simulink library "lib_imuCal"  (Simulink 9.0)
settings: Solver=VariableStepAuto  StartTime=0.0  StopTime=10.0  RelTol=1e-3
undefined symbols (not defined in the file): g, toa_imuBasicOrient
libraries: lib_CATutils_Utilities_ApplyName_v2 x14, lib_imuCal x2, simulink_extras x2, lib_CATutils_Override x2
(part 1 of 2)
settings Model: Creator=currisd  LastModifiedBy=CurriSD

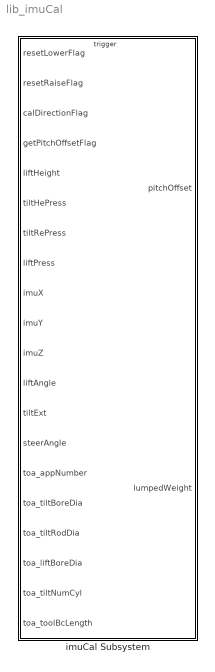
== system lib_imuCal ==
  imuCal Subsystem : Subsystem

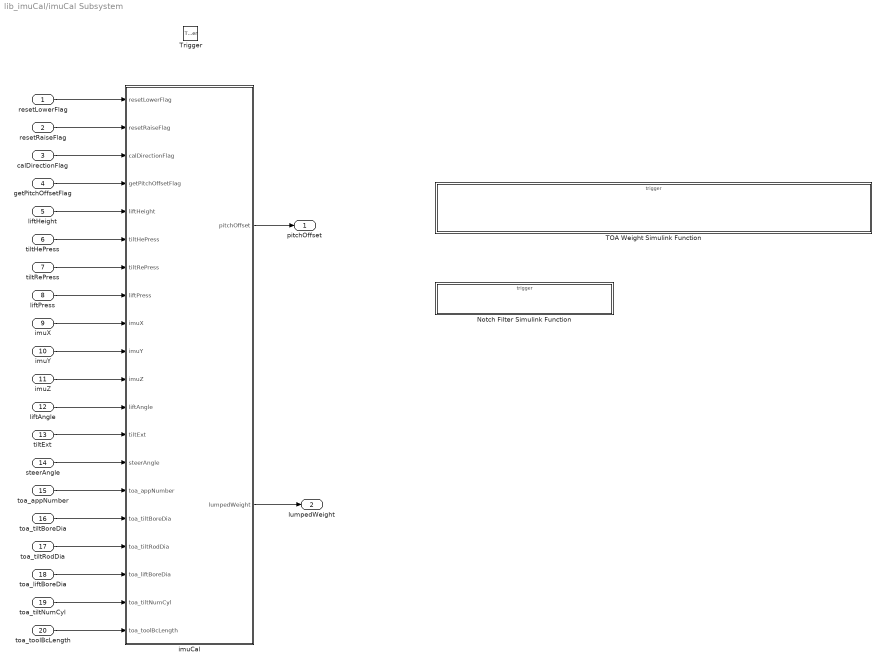
== system lib_imuCal/imuCal Subsystem ==
  resetLowerFlag : Inport
  resetRaiseFlag : Inport  Port=2
  calDirectionFlag : Inport  Port=3
  getPitchOffsetFlag : Inport  Port=4
  liftHeight : Inport  Port=5
  tiltHePress : Inport  Port=6
  tiltRePress : Inport  Port=7
  liftPress : Inport  Port=8
  imuX : Inport  Port=9
  imuY : Inport  Port=10
  imuZ : Inport  Port=11
  liftAngle : Inport  Port=12
  tiltExt : Inport  Port=13
  steerAngle : Inport  Port=14
  toa_appNumber : Inport  Port=15
  toa_tiltBoreDia : Inport  Port=16
  toa_tiltRodDia : Inport  Port=17
  toa_liftBoreDia : Inport  Port=18
  toa_tiltNumCyl : Inport  Port=19
  toa_toolBcLength : Inport  Port=20
  Trigger : TriggerPort  TriggerType=function-call  FunctionName=imuCalWrapper  FunctionVisibility=scoped  VariantControl=Variant  PortDimensions=1
  Notch Filter Simulink Function : Subsystem
  TOA Weight Simulink Function : Subsystem  TreatAsAtomicUnit=on
      settings: PropExecContextOutsideSubsystem=on
  imuCal : MATLAB Function  TreatAsAtomicUnit=on
  pitchOffset : Outport
  lumpedWeight : Outport  Port=2
  wires:
  tiltHePress/1 -> imuCal/6(tiltHePress)
  steerAngle/1 -> imuCal/14(steerAngle)
  liftHeight/1 -> imuCal/5(liftHeight)
  tiltRePress/1 -> imuCal/7(tiltRePress)
  liftPress/1 -> imuCal/8(liftPress)
  tiltExt/1 -> imuCal/13(tiltExt)
  imuZ/1 -> imuCal/11(imuZ)
  liftAngle/1 -> imuCal/12(liftAngle)
  imuX/1 -> imuCal/9(imuX)
  imuY/1 -> imuCal/10(imuY)
  resetLowerFlag/1 -> imuCal/1(resetLowerFlag)
  calDirectionFlag/1 -> imuCal/3(calDirectionFlag)
  resetRaiseFlag/1 -> imuCal/2(resetRaiseFlag)
  getPitchOffsetFlag/1 -> imuCal/4(getPitchOffsetFlag)
  imuCal/1(pitchOffset) -> pitchOffset/1
  toa_appNumber/1 -> imuCal/15(toa_appNumber)
  toa_tiltBoreDia/1 -> imuCal/16(toa_tiltBoreDia)
  toa_tiltRodDia/1 -> imuCal/17(toa_tiltRodDia)
  toa_liftBoreDia/1 -> imuCal/18(toa_liftBoreDia)
  toa_tiltNumCyl/1 -> imuCal/19(toa_tiltNumCyl)
  toa_toolBcLength/1 -> imuCal/20(toa_toolBcLength)
  imuCal/2(lumpedWeight) -> lumpedWeight/1

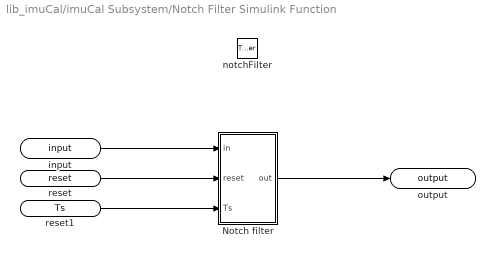
== system lib_imuCal/imuCal Subsystem/Notch Filter Simulink Function ==
  notchFilter : TriggerPort  TriggerType=function-call  IsSimulinkFunction=on  FunctionName=notchFilter  FunctionVisibility=scoped  VariantControl=Variant  PortDimensions=1
  Notch filter : Subsystem
  input : ArgIn  OutDataTypeStr=single  ArgumentName=input
  reset : ArgIn  Port=2  OutDataTypeStr=boolean  ArgumentName=reset
  reset1 : ArgIn  Port=3  OutDataTypeStr=single  ArgumentName=Ts
  output : ArgOut  OutDataTypeStr=single  ArgumentName=output
  wires:
  input/1 -> Notch filter/1(in)
  reset/1 -> Notch filter/2(reset)
  Notch filter/1(out) -> output/1
  reset1/1 -> Notch filter/3(Ts)

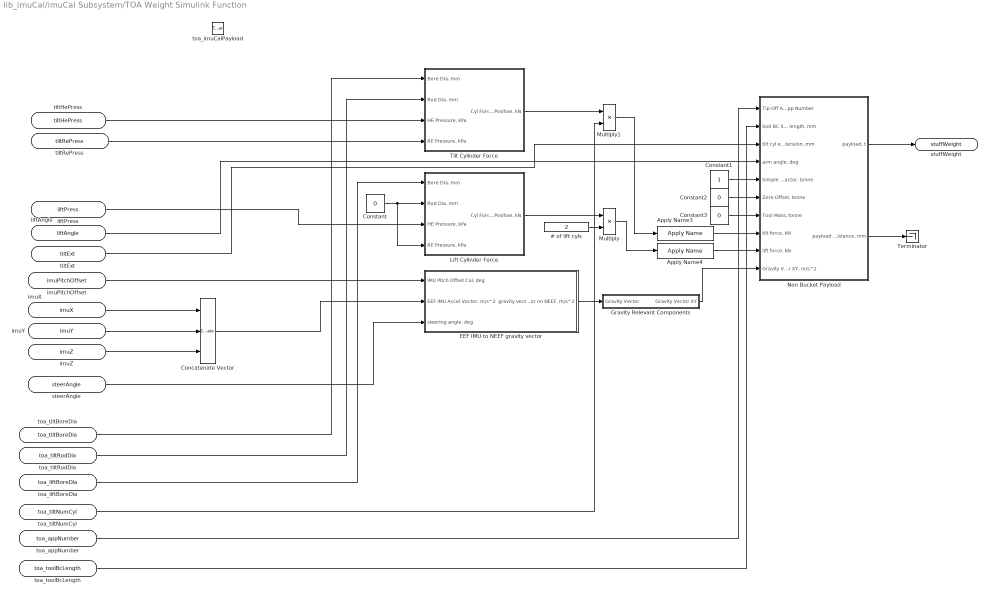
== system lib_imuCal/imuCal Subsystem/TOA Weight Simulink Function ==
  toa_imuCalPayload : TriggerPort  TriggerType=function-call  IsSimulinkFunction=on  FunctionName=toa_imuCalPayload  FunctionVisibility=scoped  VariantControl=(inherit)
  # of lift cyls : Constant  Value=2  OutDataTypeStr=single
  Apply Name3 : lib_CATutils_Utilities_ApplyName_v2/Apply Name  sigLabel='toa_tiltForce'  enTst=true
  Apply Name4 : lib_CATutils_Utilities_ApplyName_v2/Apply Name  sigLabel='toa_liftForce'  enTst=true
  Concatenate Vector : Concatenate  NumInputs=3  Mode=Multidimensional array
  Constant : Constant  Value=0  OutDataTypeStr=Inherit: Inherit via back propagation
  Constant1 : Constant  OutDataTypeStr=single
  Constant2 : Constant  Value=0  OutDataTypeStr=Inherit: Inherit via back propagation
  Constant3 : Constant  Value=0  OutDataTypeStr=Inherit: Inherit via back propagation
  EEF IMU to NEEF gravity vector : Subsystem
  Gravity Relevant Components : Subsystem
  Lift Cylinder Force : Subsystem
  Multiply : Product  SaturateOnIntegerOverflow=on  RndMeth=Zero  InputSameDT=on  OutDataTypeStr=Inherit: Same as first input
  Multiply1 : Product  OutDataTypeStr=single  SaturateOnIntegerOverflow=on  RndMeth=Zero
  Non Bucket Payload : Subsystem
  Terminator : Terminator
  Tilt Cylinder Force : Subsystem
  liftAngle : ArgIn  DisableCoverage=on  OutDataTypeStr=single  ArgumentName=liftAngle
  tiltExt : ArgIn  DisableCoverage=on  Port=2  OutDataTypeStr=single  ArgumentName=tiltExt
  tiltHePress : ArgIn  DisableCoverage=on  Port=3  OutDataTypeStr=single  ArgumentName=tiltHePress
  tiltRePress : ArgIn  DisableCoverage=on  Port=4  OutDataTypeStr=single  ArgumentName=tiltRePress
  liftPress : ArgIn  DisableCoverage=on  Port=5  OutDataTypeStr=single  ArgumentName=liftPress
  imuX : ArgIn  DisableCoverage=on  Port=6  OutDataTypeStr=single  ArgumentName=imuX
  imuY : ArgIn  DisableCoverage=on  Port=7  OutDataTypeStr=single  ArgumentName=imuY
  imuZ : ArgIn  DisableCoverage=on  Port=8  OutDataTypeStr=single  ArgumentName=imuZ
  steerAngle : ArgIn  DisableCoverage=on  Port=9  OutDataTypeStr=single  ArgumentName=steerAngle
  imuPitchOffset : ArgIn  Port=10  OutDataTypeStr=single  ArgumentName=imuPitchOffset
  toa_appNumber : ArgIn  Port=11  OutDataTypeStr=uint32  ArgumentName=toa_appNumber
  toa_tiltBoreDia : ArgIn  Port=12  OutDataTypeStr=single  ArgumentName=toa_tiltBoreDia
  toa_tiltRodDia : ArgIn  Port=13  OutDataTypeStr=single  ArgumentName=toa_tiltRodDia
  toa_liftBoreDia : ArgIn  Port=14  OutDataTypeStr=single  ArgumentName=toa_liftBoreDia
  toa_tiltNumCyl : ArgIn  Port=15  OutDataTypeStr=uint8  ArgumentName=toa_tiltNumCyl
  toa_toolBcLength : ArgIn  Port=16  OutDataTypeStr=single  ArgumentName=toa_toolBcLength
  stuffWeight : ArgOut  DisableCoverage=on  OutDataTypeStr=single  ArgumentName=stuffWeight
  wires:
  Constant2/1 -> Non Bucket Payload/6("Zero Offset, tonne")
  toa_appNumber/1 -> Non Bucket Payload/1(Tip-Off Assist App Number)
  Multiply/1 -> Apply Name4/1
  Multiply1/1 -> Apply Name3/1
  liftAngle/1 -> Non Bucket Payload/4("arm angle, deg")
  # of lift cyls/1 -> Multiply/2
  Constant/1 -> Lift Cylinder Force/4("RE Pressure, kPa"), Lift Cylinder Force/2("Rod Dia, mm")
  Constant1/1 -> Non Bucket Payload/5("Simple Cal Factor, tonne")
  Tilt Cylinder Force/1("Cyl Force, Compression Positive, kN") -> Multiply1/1
  Lift Cylinder Force/1("Cyl Force, Compression Positive, kN") -> Multiply/1
  Apply Name3/1 -> Non Bucket Payload/8("tilt force, kN")
  Apply Name4/1 -> Non Bucket Payload/9("lift force, kN")
  Constant3/1 -> Non Bucket Payload/7("Tool Mass, tonne")
  toa_tiltNumCyl/1 -> Multiply1/2
  Gravity Relevant Components/1(Gravity Vector XY) -> Non Bucket Payload/10("Gravity Vector XY, m/s^2")
  EEF IMU to NEEF gravity vector/1("gravity vector on NEEF, m/s^2") -> Gravity Relevant Components/1(Gravity Vector)
  tiltExt/1 -> Non Bucket Payload/3("tilt cyl extension, mm")
  toa_toolBcLength/1 -> Non Bucket Payload/2("tool BC link length, mm")
  Non Bucket Payload/1("payload, t") -> stuffWeight/1
  Non Bucket Payload/2("payload distance, mm") -> Terminator/1
  toa_tiltBoreDia/1 -> Tilt Cylinder Force/1("Bore Dia, mm")
  toa_tiltRodDia/1 -> Tilt Cylinder Force/2("Rod Dia, mm")
  toa_liftBoreDia/1 -> Lift Cylinder Force/1("Bore Dia, mm")
  tiltHePress/1 -> Tilt Cylinder Force/3("HE Pressure, kPa")
  tiltRePress/1 -> Tilt Cylinder Force/4("RE Pressure, kPa")
  liftPress/1 -> Lift Cylinder Force/3("HE Pressure, kPa")
  imuPitchOffset/1 -> EEF IMU to NEEF gravity vector/1("IMU Pitch Offset Cal, deg")
  Concatenate Vector/1 -> EEF IMU to NEEF gravity vector/2("EEF IMU Accel Vector, m/s^2")
  imuX/1 -> Concatenate Vector/1
  imuY/1 -> Concatenate Vector/2
  imuZ/1 -> Concatenate Vector/3
  steerAngle/1 -> EEF IMU to NEEF gravity vector/3("steering angle, deg")

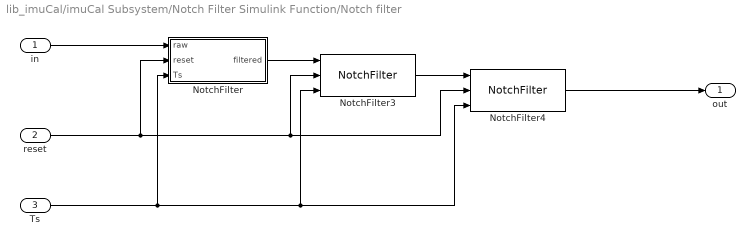
== system lib_imuCal/imuCal Subsystem/Notch Filter Simulink Function/Notch filter ==
  in : Inport
  reset : Inport  Port=2
  Ts : Inport  Port=3
  NotchFilter : Subsystem  mask{mskCutoffFreqRadPerSec=5.0}
      mask prompts: mskCutoffFreqRadPerSec "Cutoff Frequency (rad/s)"
      settings: AttributesFormatString=cf: %<mskCutoffFreqRadPerSec>
  NotchFilter3 : lib_imuCal/imuCal Subsystem/Notch Filter Simulink Function/Notch filter/NotchFilter  mskCutoffFreqRadPerSec=7.5
      settings: AttributesFormatString=cf: %<mskCutoffFreqRadPerSec>
  NotchFilter4 : lib_imuCal/imuCal Subsystem/Notch Filter Simulink Function/Notch filter/NotchFilter  mskCutoffFreqRadPerSec=12
      settings: AttributesFormatString=cf: %<mskCutoffFreqRadPerSec>
  out : Outport
  wires:
  NotchFilter/1(filtered) -> NotchFilter3/1
  NotchFilter3/1 -> NotchFilter4/1
  reset/1 -> NotchFilter3/2, NotchFilter4/2, NotchFilter/2(reset)
  in/1 -> NotchFilter/1(raw)
  NotchFilter4/1 -> out/1
  Ts/1 -> NotchFilter/3(Ts), NotchFilter4/3, NotchFilter3/3

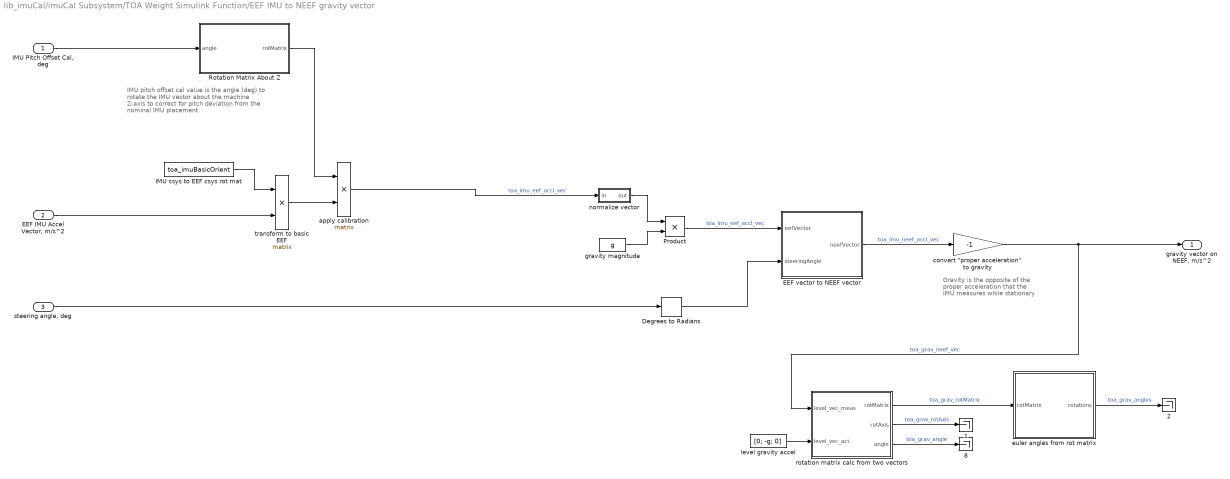
== system lib_imuCal/imuCal Subsystem/TOA Weight Simulink Function/EEF IMU to NEEF gravity vector ==
  note: Gravity is the opposite of the proper acceleration that the IMU measures while stationary
  note: IMU pitch offset cal value is the angle (deg) to rotate the IMU vector about the machine Z-axis to correct for pitch deviation from the nominal IMU placement.
  "IMU Pitch Offset Cal, deg" : Inport
  "EEF IMU Accel Vector, m/s^2" : Inport  Port=2
  "steering angle, deg" : Inport  Port=3
  " 1" : Terminator
  " 2" : Terminator
  " 8" : Terminator
  Degrees to Radians : simulink_extras/Transformations/Degrees to Radians
  EEF vector to NEEF vector : MATLAB Function  TreatAsAtomicUnit=on
  IMU csys to EEF csys rot mat : Constant  Value=toa_imuBasicOrient  VectorParams1D=off  OutDataTypeStr=single  SampleTime=-1
  Product : Product  Inputs=**  OutDataTypeStr=Inherit: Same as first input
  Rotation Matrix About Z : MATLAB Function  TreatAsAtomicUnit=on
  apply calibration : Product  Multiplication=Matrix(*)  SaturateOnIntegerOverflow=on  RndMeth=Zero  OutDataTypeStr=Inherit: Same as first input
  "convert \"proper acceleration\" to gravity" : Gain  Gain=-1  SaturateOnIntegerOverflow=on  OutDataTypeStr=Inherit: Same as input  ParamDataTypeStr=Inherit: Same as input
  euler angles from rot matrix : MATLAB Function  TreatAsAtomicUnit=on
  gravity magnitude : Constant  Value=g  OutDataTypeStr=single  SampleTime=-1
  level gravity accel : Constant  Value=[0; -g; 0]  OutDataTypeStr=single  SampleTime=-1
  normalize vector : Subsystem
  rotation matrix calc from two vectors : MATLAB Function  TreatAsAtomicUnit=on
  transform to basic EEF : Product  Multiplication=Matrix(*)  SaturateOnIntegerOverflow=on  RndMeth=Zero  OutDataTypeStr=Inherit: Same as first input
  "gravity vector on NEEF, m/s^2" : Outport
  wires:
  euler angles from rot matrix/1(rotations) -> " 2"/1  "toa_grav_angles"
  Degrees to Radians/1 -> EEF vector to NEEF vector/2(steeringAngle)
  Product/1 -> EEF vector to NEEF vector/1(eefVector)  "toa_imu_eef_accl_vec"
  "steering angle, deg"/1 -> Degrees to Radians/1
  EEF vector to NEEF vector/1(neefVector) -> "convert \"proper acceleration\" to gravity"/1  "toa_imu_neef_accl_vec"
  normalize vector/1(out) -> Product/1
  gravity magnitude/1 -> Product/2
  "IMU Pitch Offset Cal, deg"/1 -> Rotation Matrix About Z/1(angle)
  Rotation Matrix About Z/1(rotMatrix) -> apply calibration/1
  apply calibration/1 -> normalize vector/1(in)  "toa_imu_eef_accl_vec"
  transform to basic EEF/1 -> apply calibration/2
  IMU csys to EEF csys rot mat/1 -> transform to basic EEF/1
  "convert \"proper acceleration\" to gravity"/1 -> rotation matrix calc from two vectors/1(level_vec_meas), "gravity vector on NEEF, m/s^2"/1  "toa_grav_neef_vec"
  "EEF IMU Accel Vector, m/s^2"/1 -> transform to basic EEF/2
  rotation matrix calc from two vectors/1(rotMatrix) -> euler angles from rot matrix/1(rotMatrix)  "toa_grav_rotMatrix"
  rotation matrix calc from two vectors/2(rotAxis) -> " 1"/1  "toa_grav_rotAxis"
  rotation matrix calc from two vectors/3(angle) -> " 8"/1  "toa_grav_angle"
  level gravity accel/1 -> rotation matrix calc from two vectors/2(level_vec_act)

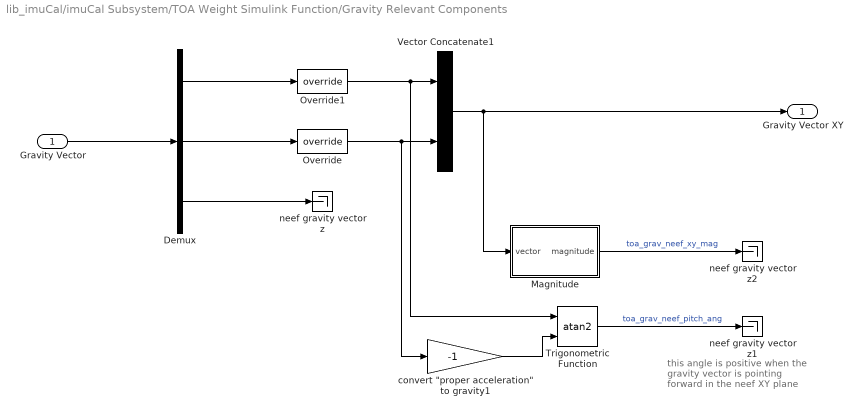
== system lib_imuCal/imuCal Subsystem/TOA Weight Simulink Function/Gravity Relevant Components ==
  note: this angle is positive when the gravity vector is pointing forward in the neef XY plane
  Gravity Vector : Inport
  " neef gravity vector z" : Terminator
  " neef gravity vector z1" : Terminator
  " neef gravity vector z2" : Terminator
  Demux : Demux  Outputs=3
  Magnitude : Subsystem
  Override : lib_CATutils_Override/override  ovType=OV if OV ~= Pass  extOV=off  ov_value=toa_grav_y_ov_val  extPass=off  pass_value=0  extRange=off  ov_max=100  ov_min=1  extCond=off  ov_cond=0  extTF=off  ov_TrueComp=1  ov_FalseComp=2
  Override1 : lib_CATutils_Override/override  ovType=OV if OV ~= Pass  extOV=off  ov_value=toa_grav_x_ov_val  extPass=off  pass_value=0  extRange=off  ov_max=100  ov_min=1  extCond=off  ov_cond=0  extTF=off  ov_TrueComp=1  ov_FalseComp=2
  Trigonometric Function : Trigonometry  Operator=atan2  OutputSignalType=real
  Vector Concatenate1 : Concatenate  Mode=Multidimensional array
  "convert \"proper acceleration\" to gravity1" : Gain  Gain=-1  SaturateOnIntegerOverflow=on  OutDataTypeStr=Inherit: Same as input  ParamDataTypeStr=Inherit: Same as input
  Gravity Vector XY : Outport
  wires:
  Gravity Vector/1 -> Demux/1
  Override/1 -> "convert \"proper acceleration\" to gravity1"/1, Vector Concatenate1/2
  Override1/1 -> Trigonometric Function/1, Vector Concatenate1/1
  Magnitude/1(magnitude) -> " neef gravity vector z2"/1  "toa_grav_neef_xy_mag"
  Trigonometric Function/1 -> " neef gravity vector z1"/1  "toa_grav_neef_pitch_ang"
  "convert \"proper acceleration\" to gravity1"/1 -> Trigonometric Function/2
  Demux/3 -> " neef gravity vector z"/1
  Demux/2 -> Override/1
  Demux/1 -> Override1/1
  Vector Concatenate1/1 -> Magnitude/1(vector), Gravity Vector XY/1

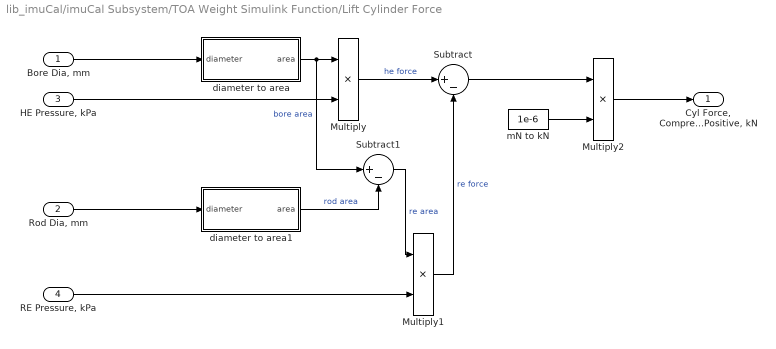
== system lib_imuCal/imuCal Subsystem/TOA Weight Simulink Function/Lift Cylinder Force ==
  "Bore Dia, mm" : Inport
  "Rod Dia, mm" : Inport  Port=2
  "HE Pressure, kPa" : Inport  Port=3
  "RE Pressure, kPa" : Inport  Port=4
  Multiply : Product  SaturateOnIntegerOverflow=on  RndMeth=Zero  InputSameDT=on  OutDataTypeStr=Inherit: Same as first input
  Multiply1 : Product  SaturateOnIntegerOverflow=on  RndMeth=Zero  InputSameDT=on  OutDataTypeStr=Inherit: Same as first input
  Multiply2 : Product  SaturateOnIntegerOverflow=on  RndMeth=Zero  InputSameDT=on  OutDataTypeStr=Inherit: Same as first input
  Subtract : Sum  Inputs=|+-  SaturateOnIntegerOverflow=on  InputSameDT=on  OutDataTypeStr=Inherit: Same as first input
  Subtract1 : Sum  Inputs=|+-  SaturateOnIntegerOverflow=on  InputSameDT=on  OutDataTypeStr=Inherit: Same as first input
  diameter to area : Subsystem
  diameter to area1 : Subsystem
  mN to kN : Constant  Value=1e-6  OutDataTypeStr=single
  "Cyl Force, Compression Positive, kN" : Outport
  wires:
  "HE Pressure, kPa"/1 -> Multiply/2
  Subtract/1 -> Multiply2/1
  "Bore Dia, mm"/1 -> diameter to area/1(diameter)
  Multiply1/1 -> Subtract/2  "re force"
  Multiply/1 -> Subtract/1  "he force"
  diameter to area/1(area) -> Subtract1/1, Multiply/1  "bore area"
  diameter to area1/1(area) -> Subtract1/2  "rod area"
  "RE Pressure, kPa"/1 -> Multiply1/2
  "Rod Dia, mm"/1 -> diameter to area1/1(diameter)
  Subtract1/1 -> Multiply1/1  "re area"
  mN to kN/1 -> Multiply2/2
  Multiply2/1 -> "Cyl Force, Compression Positive, kN"/1

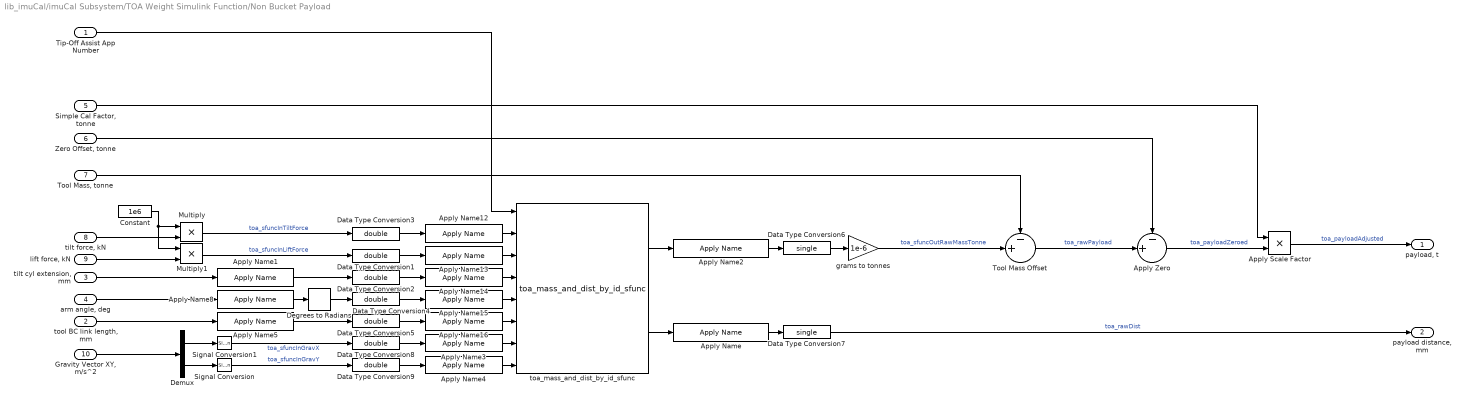
== system lib_imuCal/imuCal Subsystem/TOA Weight Simulink Function/Non Bucket Payload ==
  Tip-Off Assist App Number : Inport
  "tool BC link length, mm" : Inport  Port=2
  "tilt cyl extension, mm" : Inport  Port=3
  "arm angle, deg" : Inport  Port=4
  "Simple Cal Factor, tonne" : Inport  Port=5
  "Zero Offset, tonne" : Inport  Port=6
  "Tool Mass, tonne" : Inport  Port=7
  "tilt force, kN" : Inport  Port=8
  "lift force, kN" : Inport  Port=9
  "Gravity Vector XY, m/s^2" : Inport  Port=10
  Apply Name : lib_CATutils_Utilities_ApplyName_v2/Apply Name  sigLabel='toa_sfuncOutRawDist'  enTst=true
  Apply Name1 : lib_CATutils_Utilities_ApplyName_v2/Apply Name  sigLabel='toa_sfuncInTiltExt'  enTst=true
  Apply Name12 : lib_CATutils_Utilities_ApplyName_v2/Apply Name  sigLabel='toa_sfuncInRawTiltForce'  enTst=true
  Apply Name13 : lib_CATutils_Utilities_ApplyName_v2/Apply Name  sigLabel='toa_sfuncInRawLiftForce'  enTst=true
  Apply Name14 : lib_CATutils_Utilities_ApplyName_v2/Apply Name  sigLabel='toa_sfuncInRawTiltExt'  enTst=true
  Apply Name15 : lib_CATutils_Utilities_ApplyName_v2/Apply Name  sigLabel='toa_sfuncInRawLiftAng'  enTst=true
  Apply Name16 : lib_CATutils_Utilities_ApplyName_v2/Apply Name  sigLabel='toa_sfuncInRawBcLength'  enTst=true
  Apply Name2 : lib_CATutils_Utilities_ApplyName_v2/Apply Name  sigLabel='toa_sfuncOutRawMass'  enTst=true
  Apply Name3 : lib_CATutils_Utilities_ApplyName_v2/Apply Name  sigLabel='toa_sfuncInRawGravX'  enTst=true
  Apply Name4 : lib_CATutils_Utilities_ApplyName_v2/Apply Name  sigLabel='toa_sfuncInRawGravY'  enTst=true
  Apply Name5 : lib_CATutils_Utilities_ApplyName_v2/Apply Name  sigLabel='toa_sfuncInBcLength'  enTst=true
  Apply Name8 : lib_CATutils_Utilities_ApplyName_v2/Apply Name  sigLabel='toa_sfuncInLiftAng'  enTst=true
  Apply Scale Factor : Product
  Apply Zero : Sum  Inputs=-+|  SaturateOnIntegerOverflow=on  InputSameDT=on  OutDataTypeStr=Inherit: Same as first input
  Constant : Constant  Value=1e6  OutDataTypeStr=single
  Data Type Conversion{1..5,8..9} (7 alike) : DataTypeConversion  OutDataTypeStr=double  SaturateOnIntegerOverflow=on  RndMeth=Zero
      settings: AttributesFormatString=Output Data Type: %<OutDataTypeStr>\n
  Data Type Conversion6 : DataTypeConversion  OutDataTypeStr=single  SaturateOnIntegerOverflow=on  RndMeth=Zero
      settings: AttributesFormatString=Output Data Type: %<OutDataTypeStr>\n
  Data Type Conversion7 : DataTypeConversion  OutDataTypeStr=single  SaturateOnIntegerOverflow=on  RndMeth=Zero
      settings: AttributesFormatString=Output Data Type: %<OutDataTypeStr>\n
  Degrees to Radians : simulink_extras/Transformations/Degrees to Radians
  Demux : Demux  Outputs=2
  Multiply : Product  SaturateOnIntegerOverflow=on  RndMeth=Zero  InputSameDT=on  OutDataTypeStr=Inherit: Same as first input
  Multiply1 : Product  SaturateOnIntegerOverflow=on  RndMeth=Zero  InputSameDT=on  OutDataTypeStr=Inherit: Same as first input
  Signal Conversion : SignalConversion  OverrideOpt=on
  Signal Conversion1 : SignalConversion  OverrideOpt=on
  Tool Mass Offset : Sum  Inputs=-+|  SaturateOnIntegerOverflow=on  InputSameDT=on  OutDataTypeStr=Inherit: Same as first input
  grams to tonnes : Gain  Gain=1e-6  SaturateOnIntegerOverflow=on  OutDataTypeStr=Inherit: Same as input  ParamDataTypeStr=Inherit: Same as input
  toa_mass_and_dist_by_id_sfunc : S-Function  FunctionName=toa_mass_and_dist_by_id_sfunc  SFunctionDeploymentMode=off  EnableBusSupport=off  mask(Legacy Function){SFunctionSpec=void toa_mass_and_dist_by_id(uint32 u1, double u2, double u3, double u4, double u5, double u6, double u7, double u8, double y1[1], double y2[1]), ShowSpec=off}
      mask prompts: ShowSpec "Display function specification"
      mask help:
      | This block allows you to call the legacy functions specified by the following Legacy Code Tool definition:
      | def.SFunctionName = 'toa_mass_and_dist_by_id_sfunc';
      | def.OutputFcnSpec = 'void toa_mass_and_dist_by_id(uint32 u1, double u2, double u3, double u4, double u5, double u6, double u7, double u8, double y1[1], double y2[1])';
      | def.HeaderFiles = {'tipoff_assist.h'};
      | def.SourceFiles = {'tipoff_assist.c'};
      | def.IncPaths = {'./c_src'};
      mask Help: <p>This block was generated automatically by the Legacy Code Tool. For detailed help on this tool, call<a href="matlab:legacy_code('help')"> legacy_code('help')</a>.</p>
      mask Callback ShowSpec:
      | if strcmp(get_param(gcbh, 'ShowSpec'), 'on')
      |   set_param(gcbh, 'MaskDisplay', sprintf('fprintf(''%s'');', get_param(gcbh, 'SFunctionSpec')));
      | else
      |   set_param(gcbh, 'MaskDisplay', sprintf('fprintf(''%s'');', get_param(gcbh, 'FunctionName')));
      | end
      mask Display: fprintf('toa_mass_and_dist_by_id_sfunc');
  "payload, t" : Outport
  "payload distance, mm" : Outport  Port=2
  wires:
  Signal Conversion1/1 -> Data Type Conversion8/1  "toa_sfuncInGravX"
  Signal Conversion/1 -> Data Type Conversion9/1  "toa_sfuncInGravY"
  Apply Name1/1 -> Data Type Conversion2/1
  Apply Scale Factor/1 -> "payload, t"/1  "toa_payloadAdjusted"
  Apply Zero/1 -> Apply Scale Factor/2  "toa_payloadZeroed"
  "Simple Cal Factor, tonne"/1 -> Apply Scale Factor/1
  "Zero Offset, tonne"/1 -> Apply Zero/1
  Tool Mass Offset/1 -> Apply Zero/2  "toa_rawPayload"
  Apply Name12/1 -> toa_mass_and_dist_by_id_sfunc/2
  Apply Name13/1 -> toa_mass_and_dist_by_id_sfunc/3
  Apply Name14/1 -> toa_mass_and_dist_by_id_sfunc/4
  Apply Name15/1 -> toa_mass_and_dist_by_id_sfunc/5
  Apply Name16/1 -> toa_mass_and_dist_by_id_sfunc/6
  Apply Name3/1 -> toa_mass_and_dist_by_id_sfunc/7
  Apply Name4/1 -> toa_mass_and_dist_by_id_sfunc/8
  Tip-Off Assist App Number/1 -> toa_mass_and_dist_by_id_sfunc/1
  toa_mass_and_dist_by_id_sfunc/1 -> Apply Name2/1
  toa_mass_and_dist_by_id_sfunc/2 -> Apply Name/1
  "tilt force, kN"/1 -> Multiply/2
  "lift force, kN"/1 -> Multiply1/2
  "tool BC link length, mm"/1 -> Apply Name5/1
  Constant/1 -> Multiply1/1, Multiply/1
  Data Type Conversion3/1 -> Apply Name12/1
  Data Type Conversion1/1 -> Apply Name13/1
  Data Type Conversion2/1 -> Apply Name14/1
  Data Type Conversion4/1 -> Apply Name15/1
  Data Type Conversion5/1 -> Apply Name16/1
  Data Type Conversion6/1 -> grams to tonnes/1
  Data Type Conversion7/1 -> "payload distance, mm"/1  "toa_rawDist"
  Data Type Conversion8/1 -> Apply Name3/1
  Data Type Conversion9/1 -> Apply Name4/1
  "Tool Mass, tonne"/1 -> Tool Mass Offset/1
  "Gravity Vector XY, m/s^2"/1 -> Demux/1
  grams to tonnes/1 -> Tool Mass Offset/2  "toa_sfuncOutRawMassTonne"
  Apply Name/1 -> Data Type Conversion7/1
  Apply Name2/1 -> Data Type Conversion6/1
  Apply Name5/1 -> Data Type Conversion5/1
  Demux/2 -> Signal Conversion/1
  Demux/1 -> Signal Conversion1/1
  "tilt cyl extension, mm"/1 -> Apply Name1/1
  Multiply1/1 -> Data Type Conversion1/1  "toa_sfuncInLiftForce"
  Multiply/1 -> Data Type Conversion3/1  "toa_sfuncInTiltForce"
  Apply Name8/1 -> Degrees to Radians/1
  Degrees to Radians/1 -> Data Type Conversion4/1
  "arm angle, deg"/1 -> Apply Name8/1

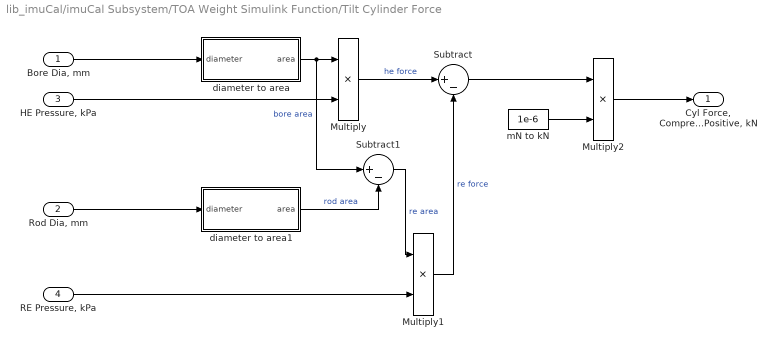
== system lib_imuCal/imuCal Subsystem/TOA Weight Simulink Function/Tilt Cylinder Force ==
  "Bore Dia, mm" : Inport
  "Rod Dia, mm" : Inport  Port=2
  "HE Pressure, kPa" : Inport  Port=3
  "RE Pressure, kPa" : Inport  Port=4
  Multiply : Product  SaturateOnIntegerOverflow=on  RndMeth=Zero  InputSameDT=on  OutDataTypeStr=Inherit: Same as first input
  Multiply1 : Product  SaturateOnIntegerOverflow=on  RndMeth=Zero  InputSameDT=on  OutDataTypeStr=Inherit: Same as first input
  Multiply2 : Product  SaturateOnIntegerOverflow=on  RndMeth=Zero  InputSameDT=on  OutDataTypeStr=Inherit: Same as first input
  Subtract : Sum  Inputs=|+-  SaturateOnIntegerOverflow=on  InputSameDT=on  OutDataTypeStr=Inherit: Same as first input
  Subtract1 : Sum  Inputs=|+-  SaturateOnIntegerOverflow=on  InputSameDT=on  OutDataTypeStr=Inherit: Same as first input
  diameter to area : Subsystem
  diameter to area1 : Subsystem
  mN to kN : Constant  Value=1e-6  OutDataTypeStr=single
  "Cyl Force, Compression Positive, kN" : Outport
  wires:
  "HE Pressure, kPa"/1 -> Multiply/2
  Subtract/1 -> Multiply2/1
  "Bore Dia, mm"/1 -> diameter to area/1(diameter)
  Multiply1/1 -> Subtract/2  "re force"
  Multiply/1 -> Subtract/1  "he force"
  diameter to area/1(area) -> Subtract1/1, Multiply/1  "bore area"
  diameter to area1/1(area) -> Subtract1/2  "rod area"
  "RE Pressure, kPa"/1 -> Multiply1/2
  "Rod Dia, mm"/1 -> diameter to area1/1(diameter)
  Subtract1/1 -> Multiply1/1  "re area"
  mN to kN/1 -> Multiply2/2
  Multiply2/1 -> "Cyl Force, Compression Positive, kN"/1

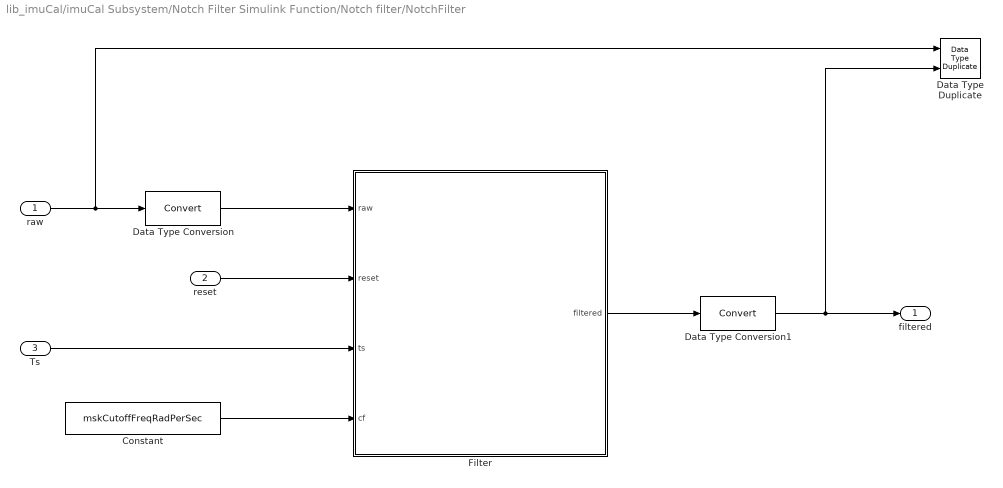
== system lib_imuCal/imuCal Subsystem/Notch Filter Simulink Function/Notch filter/NotchFilter ==
  raw : Inport
  reset : Inport  Port=2
  Ts : Inport  Port=3
  Constant : Constant  Value=mskCutoffFreqRadPerSec  OutDataTypeStr=Inherit: Inherit via back propagation
  Data Type Duplicate : DataTypeDuplicate
  Data Type Conversion : DataTypeConversion
  Data Type Conversion1 : DataTypeConversion  SaturateOnIntegerOverflow=on
  Filter : Stateflow chart  TreatAsAtomicUnit=on
  filtered : Outport
  wires:
  Filter/1(filtered) -> Data Type Conversion1/1
  reset/1 -> Filter/2(reset)
  Constant/1 -> Filter/4(cf)
  Data Type Conversion/1 -> Filter/1(raw)
  Data Type Conversion1/1 -> Data Type Duplicate/2, filtered/1
  raw/1 -> Data Type Duplicate/1, Data Type Conversion/1
  Ts/1 -> Filter/3(ts)

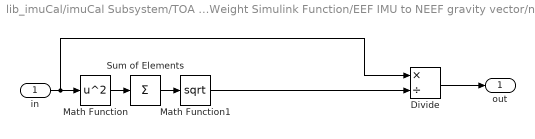
== system lib_imuCal/imuCal Subsystem/TOA Weight Simulink Function/EEF IMU to NEEF gravity vector/normalize vector ==
  in : Inport
  Divide : Product  Inputs=*/  OutDataTypeStr=Inherit: Same as first input
  Math Function : Math  Operator=square  SaturateOnIntegerOverflow=on
  Math Function1 : Math  Operator=sqrt  SaturateOnIntegerOverflow=on
  Sum of Elements : Sum  Inputs=+
  out : Outport
  wires:
  Sum of Elements/1 -> Math Function1/1
  Math Function/1 -> Sum of Elements/1
  Math Function1/1 -> Divide/2
  in/1 -> Divide/1, Math Function/1
  Divide/1 -> out/1

== system lib_imuCal/imuCal Subsystem/TOA Weight Simulink Function/Gravity Relevant Components/Magnitude ==
  vector : Inport
  Math Function : Math  Operator=square  SaturateOnIntegerOverflow=on
  Math Function1 : Math  Operator=sqrt  SaturateOnIntegerOverflow=on
  Sum of Elements : Sum  Inputs=+
  magnitude : Outport
  wires:
  Math Function1/1 -> magnitude/1
  Math Function/1 -> Sum of Elements/1
  Sum of Elements/1 -> Math Function1/1
  vector/1 -> Math Function/1

== system lib_imuCal/imuCal Subsystem/TOA Weight Simulink Function/Lift Cylinder Force/diameter to area ==
  diameter : Inport
  Constant2 : Constant  Value=pi/4  OutDataTypeStr=single
  Math Function : Math  Operator=square  OutputSignalType=real  SaturateOnIntegerOverflow=on
  Multiply2 : Product  SaturateOnIntegerOverflow=on  RndMeth=Zero  InputSameDT=on  OutDataTypeStr=Inherit: Same as first input
  area : Outport
  wires:
  Constant2/1 -> Multiply2/1
  Math Function/1 -> Multiply2/2
  Multiply2/1 -> area/1
  diameter/1 -> Math Function/1

== system lib_imuCal/imuCal Subsystem/TOA Weight Simulink Function/Lift Cylinder Force/diameter to area1 ==
  diameter : Inport
  Constant2 : Constant  Value=pi/4  OutDataTypeStr=single
  Math Function : Math  Operator=square  OutputSignalType=real  SaturateOnIntegerOverflow=on
  Multiply2 : Product  SaturateOnIntegerOverflow=on  RndMeth=Zero  InputSameDT=on  OutDataTypeStr=Inherit: Same as first input
  area : Outport
  wires:
  Constant2/1 -> Multiply2/1
  Math Function/1 -> Multiply2/2
  Multiply2/1 -> area/1
  diameter/1 -> Math Function/1

== system lib_imuCal/imuCal Subsystem/TOA Weight Simulink Function/Tilt Cylinder Force/diameter to area ==
  diameter : Inport
  Constant2 : Constant  Value=pi/4  OutDataTypeStr=single
  Math Function : Math  Operator=square  OutputSignalType=real  SaturateOnIntegerOverflow=on
  Multiply2 : Product  SaturateOnIntegerOverflow=on  RndMeth=Zero  InputSameDT=on  OutDataTypeStr=Inherit: Same as first input
  area : Outport
  wires:
  Constant2/1 -> Multiply2/1
  Math Function/1 -> Multiply2/2
  Multiply2/1 -> area/1
  diameter/1 -> Math Function/1

== system lib_imuCal/imuCal Subsystem/TOA Weight Simulink Function/Tilt Cylinder Force/diameter to area1 ==
  diameter : Inport
  Constant2 : Constant  Value=pi/4  OutDataTypeStr=single
  Math Function : Math  Operator=square  OutputSignalType=real  SaturateOnIntegerOverflow=on
  Multiply2 : Product  SaturateOnIntegerOverflow=on  RndMeth=Zero  InputSameDT=on  OutDataTypeStr=Inherit: Same as first input
  area : Outport
  wires:
  Constant2/1 -> Multiply2/1
  Math Function/1 -> Multiply2/2
  Multiply2/1 -> area/1
  diameter/1 -> Math Function/1

== stateflow chart imuCal Subsystem/Notch Filter Simulink Function/Notch filter/NotchFilter/Filter ==
  state Update
    du: updateFilter();
  state initFilter [function]
    (default) -> (junction 11) : {
        | q = (cf*cf*ts*ts)/4.0c;
        | r = cf*ts;
        | p = 1.0c + q;
        | s = 2.0c * (q - 1.0c);
        | t = p + r;
        |
        | alpha = p / t;
        | beta = s / t;
        | gamma = r / t;
        | }
    (junction 11) -> (junction 12) : {
        | rawHist[0] = raw;
        | rawHist[1] = raw;
        | rawHist[2] = raw;
        | }
    (junction 12) -> (junction 13) : {
        | filtHist[0] = raw;
        | filtHist[1] = raw;
        | filtHist[2] = raw;
        | }
    (junction 13) -> (junction 14) : {
        | filtered = filtHist[0];
        | }
  state updateFilter [function]
    (default) -> (junction 19) : {
        | rawHist[2] = rawHist[1];
        | rawHist[1] = rawHist[0];
        | rawHist[0] = raw;
        | }
    (junction 19) -> (junction 20) : {
        | filtHist[2] = filtHist[1];
        | filtHist[1] = filtHist[0];
        | filtHist[0] = (alpha * (rawHist[0] + rawHist[2] - filtHist[2])) + (beta * (rawHist[1] - filtHist[1])) + (gamma * filtHist[2]);
        | }
    (junction 20) -> (junction 21) : {
        | filtered = filtHist[0];
        | }
  (default) -> (junction 35)
  Update -> (junction 35) : [reset]
  (junction 35) -> Update : {initFilter();}
  data: q temporary single; r temporary single; p temporary single; s temporary single; t temporary single; raw input single; reset input boolean; ts input single; cf input single; filtered output single; rawHist local single size=3; filtHist local single size=3; alpha local single; beta local single; gamma local single

== matlab function imuCal Subsystem/TOA Weight Simulink Function/EEF IMU to NEEF gravity vector/Rotation Matrix About Z ==
  data: angle input double; rotMatrix output double
function rotMatrix = fcn(angle)
% Calculates a rotation matrix from an angle in deg
if angle == 0
    rotMatrix = single(eye(3));
    return
end

angleRad = angle / 180.0 * pi;

% Form rotation matrix
a = cos(angleRad);
b = sin(angleRad);
rotMatrix = [
    a, -b, 0;
    b, a, 0;
    0, 0, 1
    ];

== matlab function imuCal Subsystem/TOA Weight Simulink Function/EEF IMU to NEEF gravity vector/EEF vector to NEEF vector ==
  data: eefVector input double; neefVector output double; steeringAngle input double
function neefVector  = fcn(eefVector, steeringAngle)
% Transforms a vector on the EEF to a vector on the NEEF via steering angle
rotAxis = [0; 1; 0];               % Steering right is positive angle
angle = steeringAngle;

% Form rotation matrix
crossProductMatrix = [
    0,          -rotAxis(3),  rotAxis(2);
     rotAxis(3), 0,          -rotAxis(1);
    -rotAxis(2), rotAxis(1),  0
];
tensorProduct = rotAxis * transpose(rotAxis);
rotMatrix = cos(angle) * eye(3) + sin(angle) * crossProductMatrix + ...
    (1 - cos(angle)) * tensorProduct;

neefVector = rotMatrix * eefVector;
